simulink model "StarshipSystemModel"  (R2025b)
settings: Solver=VariableStepAuto  StartTime=0.0  StopTime=10.0  RelTol=1e-3
model workspace (MAT data in the model file):
  ActiveGNCMode : Simulink.Bus (value not decoded)
  AerodynamicControlCommand : Simulink.Bus (value not decoded)
  AerodynamicLoad : Simulink.Bus (value not decoded)
  AggregatedStream : Simulink.Bus (value not decoded)
  AllocatedEffectorDemand : Simulink.Bus (value not decoded)
  AttitudeControlDemand : Simulink.Bus (value not decoded)
  AttitudeGuidanceCommand : Simulink.Bus (value not decoded)
  AttitudeRateState : Simulink.Bus (value not decoded)
  AutogenousPressurantGas : Simulink.ConnectionBus (value not decoded)
  CandidateFaultIndication : Simulink.Bus (value not decoded)
  CombustionGasFeed : Simulink.ConnectionBus (value not decoded)
  CommandPathHealth : Simulink.Bus (value not decoded)
  ControlMode : Simulink.ValueType (value not decoded)
  DownlinkSignal : Simulink.Bus (value not decoded)
  ElectricalPower : Simulink.ConnectionBus (value not decoded)
  EngineTelemetry : Simulink.Bus (value not decoded)
  ExecutionContext : Simulink.Bus (value not decoded)
  FaultDiagnosisResult : Simulink.Bus (value not decoded)
  GNCDataContext : Simulink.Bus (value not decoded)
  GNCHealthState : Simulink.Bus (value not decoded)
  GNCStateEstimate : Simulink.Bus (value not decoded)
  GimbalAngle : Simulink.ValueType (value not decoded)
  GimbalMotion : Simulink.ConnectionBus (value not decoded)
  GroundCheckoutLink : Simulink.Bus (value not decoded)
  GroundPressurantSupply : Simulink.ConnectionBus (value not decoded)
  GuidanceConstraints : Simulink.Bus (value not decoded)
  GuidanceMode : Simulink.ValueType (value not decoded)
  LinkHealth : Simulink.Bus (value not decoded)
  LiquidPropellantFeed : Simulink.ConnectionBus (value not decoded)
  MechanicalMotion : Simulink.ConnectionBus (value not decoded)
  MechanismPosition : Simulink.Bus (value not decoded)
  ModeTransitionContext : Simulink.Bus (value not decoded)
  NavigationAidingData : Simulink.Bus (value not decoded)
  NavigationEstimate : Simulink.Bus (value not decoded)
  NavigationHealthStatus : Simulink.Bus (value not decoded)
  NavigationMeasurementSet : Simulink.Bus (value not decoded)
  PercentThrottle : Simulink.ValueType (value not decoded)
  PneumaticActuationGas : Simulink.ConnectionBus (value not decoded)
  PowerConversionStatus : Simulink.Bus (value not decoded)
  PowerDistributionStatus : Simulink.Bus (value not decoded)
  PowerHealthStatus : Simulink.Bus (value not decoded)
  PowerManagementCommand : Simulink.Bus (value not decoded)
  PowerStorageStatus : Simulink.Bus (value not decoded)
  ProtectedThermalState : Simulink.Bus (value not decoded)
  ProtectionIsolationStatus : Simulink.Bus (value not decoded)
  PurgeGasSupply : Simulink.ConnectionBus (value not decoded)
  RCSPulseCommand : Simulink.Bus (value not decoded)
  RCSTelemetry : Simulink.Bus (value not decoded)
  RFFeed : Simulink.ConnectionBus (value not decoded)
  RecoveryMechanismCommand : Simulink.Bus (value not decoded)
  RollThrottleBias : Simulink.ValueType (value not decoded)
  SafetyOverride : Simulink.ValueType (value not decoded)
  SafetyStateStatus : Simulink.Bus (value not decoded)
  ShapedControlDemand : Simulink.Bus (value not decoded)
  SpinStartIgniterGas : Simulink.ConnectionBus (value not decoded)
  StageMechanicalBoundary : Simulink.ConnectionBus (value not decoded)
  StructuralLoad : Simulink.ConnectionBus (value not decoded)
  StructureHealthStatus : Simulink.Bus (value not decoded)
  SubsystemHealthEvidence : Simulink.Bus (value not decoded)
  SubsystemStatusTelemetry : Simulink.Bus (value not decoded)
  TankTelemetry : Simulink.Bus (value not decoded)
  ThermalMonitoringCommand : Simulink.Bus (value not decoded)
  ThermalNetwork : Simulink.ConnectionBus (value not decoded)
  ThrustLoad : Simulink.ConnectionBus (value not decoded)
  TrajectoryGuidanceCommand : Simulink.Bus (value not decoded)
  TrajectoryReference : Simulink.Bus (value not decoded)
  TranslationalControlDemand : Simulink.Bus (value not decoded)
  TranslationalState : Simulink.Bus (value not decoded)
  UplinkSignal : Simulink.Bus (value not decoded)
  ValidatedControlDemand : Simulink.Bus (value not decoded)
  ValveCommand : Simulink.ValueType (value not decoded)
  VehicleStructureState : Simulink.Bus (value not decoded)
  VerifiedCommand : Simulink.Bus (value not decoded)
  VideoStream : Simulink.Bus (value not decoded)
undefined symbols (not defined in the file): ACR, ACT, ASM, ATM, BCR, BDQ, BDR, BDX, BEC, BFC, BHV, BIP, BLM, BNZ, BPI, BPR, BPV, BRX, BSM, BTA, BTP, BVC, BVE, BVV, CAA, CAM, CAS, CAT, CLM, COM, CRS, CTL, CTR, DAQ, ESC, EXT, FCR, FDB, FDE, FEX, FHI, FHM, FIC, FIS, FMG, FSC, GAP, GCM, GMD, GNC, GND, GPH, GTR, HDN, HIA, HSI, IF, INT, LOC, NAI ... (+45)
(part 2 of 8)

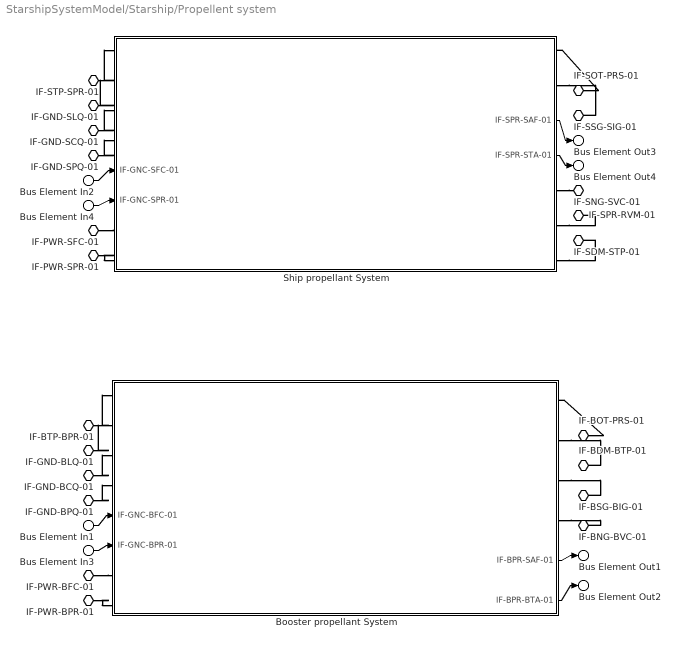
== system StarshipSystemModel/Starship/Propellent system ==
  Bus Element In1 : Inport  PortName=IF-GNC-BFC-01
  Bus Element In2 : Inport  Port=2  PortName=IF-GNC-SFC-01
  Bus Element In3 : Inport  Port=3  PortName=IF-GNC-BPR-01
  Bus Element In4 : Inport  Port=4  PortName=IF-GNC-SPR-01
  Booster propellant System : Subsystem
      settings: PortSchema="{\"entries\":[{\"content\":{\"headerSize\":26,\"margin\":15,\"minimumSpacing\":25,\"sides\":[{\"content\":{\"connectorIds\":[\"LConn2\",\"LConn3\",\"LConn4\",\"LConn7\",\"In1\",\"In2\",\"LConn5\",\"LConn6\"]},\"type\":\"ConnectorPlacement.EquallySpacedRectSide\",\"uuid\":\"fbe4f8e6-132c-4a0c-8c4c-52d0209da778\"},{\"content\":{\"connectorIds\":[\"LConn1\",\"RConn1\",\"RConn2\",\"RConn3\",\"Out1\",\"Out2\"],\"side\":\"RIGHT\"},\"type\":\"ConnectorPlacement.EquallySpacedRectSide\",\"uuid\":\"bbe80fa3-b8e3-44c5-9574-5758a55378fd\"},{\"content\":{\"side\":\"TOP\"},\"type\":\"ConnectorPlacement.EquallySpacedRectSide\",\"uuid\":\"410005e2-e10b-4d3e-a617-d51b1ea5de7e\"}]},\"type\":\"ConnectorPlacement.EquallySpacedConnector\",\"uuid\":\"b66a347a-e5b4-46b1-8a3f-28cf70f30a27\"}],\"packageUris\":[\"http://schema.mathworks.com/mf0/Connector/R2020b\"],\"version\":\"1.0\"}"
  Ship propellant System : Subsystem
      settings: PortSchema="{\"entries\":[{\"content\":{\"headerSize\":26,\"margin\":15,\"minimumSpacing\":25,\"sides\":[{\"content\":{\"connectorIds\":[\"LConn2\",\"LConn3\",\"LConn4\",\"LConn6\",\"In1\",\"In2\",\"LConn5\",\"RConn1\"]},\"type\":\"ConnectorPlacement.EquallySpacedRectSide\",\"uuid\":\"fbe4f8e6-132c-4a0c-8c4c-52d0209da778\"},{\"content\":{\"connectorIds\":[\"LConn1\",\"RConn2\",\"Out1\",\"Out2\",\"RConn3\",\"RConn4\",\"RConn5\"],\"side\":\"RIGHT\"},\"type\":\"ConnectorPlacement.EquallySpacedRectSide\",\"uuid\":\"bbe80fa3-b8e3-44c5-9574-5758a55378fd\"},{\"content\":{\"side\":\"TOP\"},\"type\":\"ConnectorPlacement.EquallySpacedRectSide\",\"uuid\":\"410005e2-e10b-4d3e-a617-d51b1ea5de7e\"},{\"content\":{\"side\":\"BOTTOM\"},\"type\":\"ConnectorPlacement.EquallySpacedRectSide\",\"uuid\":\"fc3d345f-9ee7-43d3-a8e7-80d4ac46c4c5\"}]},\"type\":\"ConnectorPlacement.EquallySpacedConnector\",\"uuid\":\"b66a347a-e5b4-46b1-8a3f-28cf70f30a27\"}],\"packageUris\":[\"http://schema.mathworks.com/mf0/Connector/R2020b\"],\"version\":\"1.0\"}"
  IF-BDM-BTP-01 : PMIOPort  Side=Right  ConnectionType=Bus: LiquidPropellantFeed
  IF-BSG-BIG-01 : PMIOPort  Port=2  Side=Right  ConnectionType=Bus: SpinStartIgniterGas
  IF-BNG-BVC-01 : PMIOPort  Port=3  Side=Right  ConnectionType=Bus: PneumaticActuationGas
  IF-SDM-STP-01 : PMIOPort  Port=4  Side=Right  ConnectionType=Bus: LiquidPropellantFeed
  IF-SPR-RVM-01 : PMIOPort  Port=5  Side=Right  ConnectionType=Bus: CombustionGasFeed
  IF-SNG-SVC-01 : PMIOPort  Port=6  Side=Right  ConnectionType=Bus: PneumaticActuationGas
  IF-SSG-SIG-01 : PMIOPort  Port=7  Side=Right  ConnectionType=Bus: SpinStartIgniterGas
  IF-BOT-PRS-01 : PMIOPort  Port=8  Side=Left  ConnectionType=Bus: StructuralLoad
  IF-SOT-PRS-01 : PMIOPort  Port=9  Side=Left  ConnectionType=Bus: StructuralLoad
  IF-BTP-BPR-01 : PMIOPort  Port=10  Side=Left  ConnectionType=Bus: AutogenousPressurantGas
  "IF-GND-BLQ-01\t" : PMIOPort  Port=11  Side=Left
  IF-STP-SPR-01 : PMIOPort  Port=12  Side=Left  ConnectionType=Bus: AutogenousPressurantGas
  "IF-GND-BCQ-01\t" : PMIOPort  Port=13  Side=Left
  IF-GND-BPQ-01 : PMIOPort  Port=14  Side=Left  ConnectionType=Bus: GroundPressurantSupply
  IF-GND-SLQ-01 : PMIOPort  Port=15  Side=Left
  IF-PWR-BFC-01 : PMIOPort  Port=16  Side=Left  ConnectionType=Bus: ElectricalPower
  IF-PWR-BPR-01 : PMIOPort  Port=17  Side=Left  ConnectionType=Bus: ElectricalPower
  IF-PWR-SFC-01 : PMIOPort  Port=18  Side=Left  ConnectionType=Bus: ElectricalPower
  IF-PWR-SPR-01 : PMIOPort  Port=19  Side=Left  ConnectionType=Bus: ElectricalPower
  IF-GND-SCQ-01 : PMIOPort  Port=20  Side=Left
  IF-GND-SPQ-01 : PMIOPort  Port=21  Side=Left  ConnectionType=Bus: GroundPressurantSupply
  Bus Element Out2 : Outport  PortName=IF-BPR-BTA-01
  Bus Element Out4 : Outport  Port=2  PortName=IF-SPR-STA-01
  Bus Element Out3 : Outport  Port=3  PortName=IF-SPR-SAF-01
  Bus Element Out1 : Outport  Port=4  PortName=IF-BPR-SAF-01
  wires:
  Booster propellant System/1(IF-BPR-SAF-01) -> Bus Element Out1/1
  Bus Element In2/1 -> Ship propellant System/1(IF-GNC-SFC-01)
  Bus Element In4/1 -> Ship propellant System/2(IF-GNC-SPR-01)
  Bus Element In3/1 -> Booster propellant System/2(IF-GNC-BPR-01)
  Bus Element In1/1 -> Booster propellant System/1(IF-GNC-BFC-01)
  Booster propellant System/2(IF-BPR-BTA-01) -> Bus Element Out2/1
  Ship propellant System/1(IF-SPR-SAF-01) -> Bus Element Out3/1
  Ship propellant System/2(IF-SPR-STA-01) -> Bus Element Out4/1
  connections:
  IF-STP-SPR-01/RConn1 -- Ship propellant System/LConn2
  IF-GND-SPQ-01/RConn1 -- Ship propellant System/LConn6
  Booster propellant System/RConn1 -- IF-BDM-BTP-01/RConn1
  IF-GND-SCQ-01/RConn1 -- Ship propellant System/LConn4
  IF-GND-SLQ-01/RConn1 -- Ship propellant System/LConn3
  IF-BTP-BPR-01/RConn1 -- Booster propellant System/LConn2
  "IF-GND-BLQ-01\t"/RConn1 -- Booster propellant System/LConn3
  "IF-GND-BCQ-01\t"/RConn1 -- Booster propellant System/LConn4
  Booster propellant System/RConn3 -- IF-BNG-BVC-01/RConn1
  IF-GND-BPQ-01/RConn1 -- Booster propellant System/LConn7
  Ship propellant System/RConn2 -- IF-SSG-SIG-01/RConn1
  Ship propellant System/RConn3 -- IF-SNG-SVC-01/RConn1
  Ship propellant System/RConn4 -- IF-SPR-RVM-01/RConn1
  Ship propellant System/RConn5 -- IF-SDM-STP-01/RConn1
  Booster propellant System/RConn2 -- IF-BSG-BIG-01/RConn1
  IF-BOT-PRS-01/RConn1 -- Booster propellant System/LConn1
  IF-SOT-PRS-01/RConn1 -- Ship propellant System/LConn1
  IF-PWR-BFC-01/RConn1 -- Booster propellant System/LConn5
  IF-PWR-BPR-01/RConn1 -- Booster propellant System/LConn6
  IF-PWR-SFC-01/RConn1 -- Ship propellant System/LConn5
  IF-PWR-SPR-01/RConn1 -- Ship propellant System/RConn1

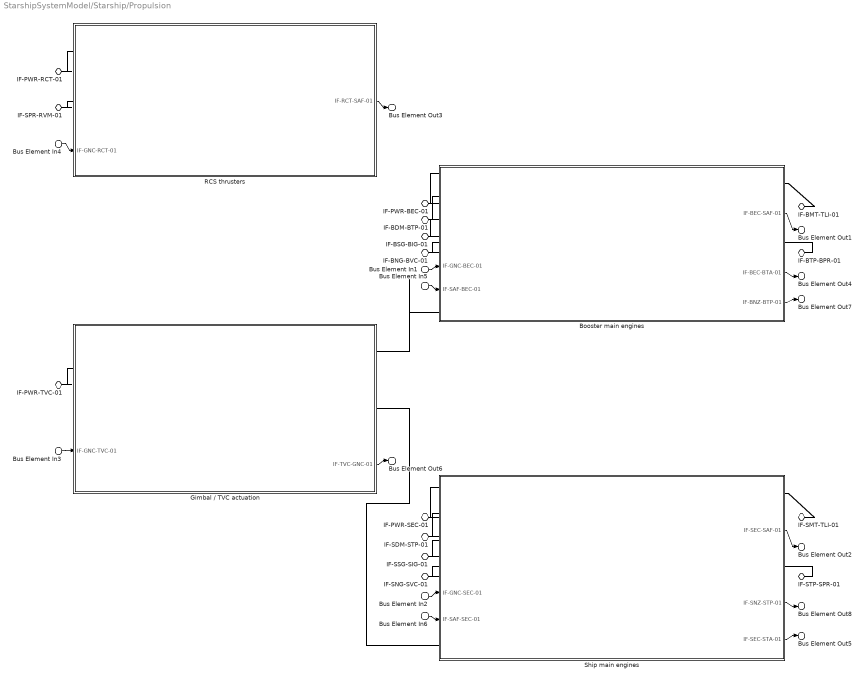
== system StarshipSystemModel/Starship/Propulsion ==
  Bus Element In1 : Inport  PortName=IF-GNC-BEC-01
  Bus Element In2 : Inport  Port=2  PortName=IF-GNC-SEC-01
  Bus Element In3 : Inport  Port=3  PortName=IF-GNC-TVC-01
  Bus Element In4 : Inport  Port=4  PortName=IF-GNC-RCT-01
  Bus Element In5 : Inport  Port=5  PortName=IF-SAF-BEC-01
  Bus Element In6 : Inport  Port=6  PortName=IF-SAF-SEC-01
  Booster main engines : Subsystem
      settings: PortSchema="{\"entries\":[{\"content\":{\"headerSize\":26,\"margin\":15,\"minimumSpacing\":25,\"sides\":[{\"content\":{\"connectorIds\":[\"LConn1\",\"LConn3\",\"LConn4\",\"LConn5\",\"In1\",\"In2\",\"LConn6\"]},\"type\":\"ConnectorPlacement.EquallySpacedRectSide\",\"uuid\":\"a24f90f9-b52e-4407-98a2-61cef3ed1001\"},{\"content\":{\"connectorIds\":[\"LConn2\",\"Out1\",\"RConn1\",\"Out2\",\"Out3\"],\"side\":\"RIGHT\"},\"type\":\"ConnectorPlacement.EquallySpacedRectSide\",\"uuid\":\"349c89d4-9966-4ad9-ba76-db4d38641e72\"},{\"content\":{\"side\":\"TOP\"},\"type\":\"ConnectorPlacement.EquallySpacedRectSide\",\"uuid\":\"c23b8a3e-5693-4bb4-96b3-90d999333c4e\"}]},\"type\":\"ConnectorPlacement.EquallySpacedConnector\",\"uuid\":\"ab682651-c32f-4460-8c4f-01dcf64563ad\"}],\"packageUris\":[\"http://schema.mathworks.com/mf0/Connector/R2020b\"],\"version\":\"1.0\"}"
  Gimbal / TVC actuation : Subsystem
      settings: PortSchema="{\"entries\":[{\"content\":{\"headerSize\":26,\"margin\":15,\"minimumSpacing\":25,\"sides\":[{\"content\":{\"connectorIds\":[\"LConn1\",\"In1\"]},\"type\":\"ConnectorPlacement.EquallySpacedRectSide\",\"uuid\":\"a24f90f9-b52e-4407-98a2-61cef3ed1001\"},{\"content\":{\"connectorIds\":[\"RConn1\",\"RConn2\",\"Out1\"],\"side\":\"RIGHT\"},\"type\":\"ConnectorPlacement.EquallySpacedRectSide\",\"uuid\":\"349c89d4-9966-4ad9-ba76-db4d38641e72\"},{\"content\":{\"side\":\"TOP\"},\"type\":\"ConnectorPlacement.EquallySpacedRectSide\",\"uuid\":\"c23b8a3e-5693-4bb4-96b3-90d999333c4e\"}]},\"type\":\"ConnectorPlacement.EquallySpacedConnector\",\"uuid\":\"ab682651-c32f-4460-8c4f-01dcf64563ad\"}],\"packageUris\":[\"http://schema.mathworks.com/mf0/Connector/R2020b\"],\"version\":\"1.0\"}"
  RCS thrusters : Subsystem
      settings: PortSchema="{\"entries\":[{\"content\":{\"headerSize\":26,\"margin\":15,\"minimumSpacing\":25,\"sides\":[{\"content\":{\"connectorIds\":[\"LConn1\",\"LConn2\",\"In1\"]},\"type\":\"ConnectorPlacement.EquallySpacedRectSide\",\"uuid\":\"a24f90f9-b52e-4407-98a2-61cef3ed1001\"},{\"content\":{\"connectorIds\":[\"Out1\"],\"side\":\"RIGHT\"},\"type\":\"ConnectorPlacement.EquallySpacedRectSide\",\"uuid\":\"349c89d4-9966-4ad9-ba76-db4d38641e72\"},{\"content\":{\"side\":\"TOP\"},\"type\":\"ConnectorPlacement.EquallySpacedRectSide\",\"uuid\":\"c23b8a3e-5693-4bb4-96b3-90d999333c4e\"}]},\"type\":\"ConnectorPlacement.EquallySpacedConnector\",\"uuid\":\"ab682651-c32f-4460-8c4f-01dcf64563ad\"}],\"packageUris\":[\"http://schema.mathworks.com/mf0/Connector/R2020b\"],\"version\":\"1.0\"}"
  Ship main engines : Subsystem
      settings: PortSchema="{\"entries\":[{\"content\":{\"headerSize\":26,\"margin\":15,\"minimumSpacing\":25,\"sides\":[{\"content\":{\"connectorIds\":[\"LConn1\",\"LConn3\",\"LConn4\",\"LConn5\",\"In1\",\"In2\",\"LConn6\"]},\"type\":\"ConnectorPlacement.EquallySpacedRectSide\",\"uuid\":\"a24f90f9-b52e-4407-98a2-61cef3ed1001\"},{\"content\":{\"connectorIds\":[\"LConn2\",\"Out1\",\"RConn1\",\"Out2\",\"Out3\"],\"side\":\"RIGHT\"},\"type\":\"ConnectorPlacement.EquallySpacedRectSide\",\"uuid\":\"349c89d4-9966-4ad9-ba76-db4d38641e72\"},{\"content\":{\"side\":\"TOP\"},\"type\":\"ConnectorPlacement.EquallySpacedRectSide\",\"uuid\":\"c23b8a3e-5693-4bb4-96b3-90d999333c4e\"}]},\"type\":\"ConnectorPlacement.EquallySpacedConnector\",\"uuid\":\"ab682651-c32f-4460-8c4f-01dcf64563ad\"}],\"packageUris\":[\"http://schema.mathworks.com/mf0/Connector/R2020b\"],\"version\":\"1.0\"}"
  IF-PWR-RCT-01 : PMIOPort  Side=Left  ConnectionType=Bus: ElectricalPower
  IF-PWR-TVC-01 : PMIOPort  Port=2  Side=Left  ConnectionType=Bus: ElectricalPower
  IF-PWR-BEC-01 : PMIOPort  Port=3  Side=Left  ConnectionType=Bus: ElectricalPower
  IF-PWR-SEC-01 : PMIOPort  Port=4  Side=Left  ConnectionType=Bus: ElectricalPower
  IF-BMT-TLI-01 : PMIOPort  Port=5  Side=Left  ConnectionType=Bus: StructuralLoad
  IF-SMT-TLI-01 : PMIOPort  Port=6  Side=Left  ConnectionType=Bus: StructuralLoad
  IF-BDM-BTP-01 : PMIOPort  Port=7  Side=Left  ConnectionType=Bus: LiquidPropellantFeed
  IF-SDM-STP-01 : PMIOPort  Port=8  Side=Left  ConnectionType=Bus: LiquidPropellantFeed
  IF-SPR-RVM-01 : PMIOPort  Port=9  Side=Left  ConnectionType=Bus: CombustionGasFeed
  IF-BSG-BIG-01 : PMIOPort  Port=10  Side=Left  ConnectionType=Bus: SpinStartIgniterGas
  IF-BNG-BVC-01 : PMIOPort  Port=11  Side=Left  ConnectionType=Bus: PneumaticActuationGas
  IF-SSG-SIG-01 : PMIOPort  Port=12  Side=Left  ConnectionType=Bus: SpinStartIgniterGas
  IF-SNG-SVC-01 : PMIOPort  Port=13  Side=Left  ConnectionType=Bus: PneumaticActuationGas
  IF-BTP-BPR-01 : PMIOPort  Port=14  Side=Right  ConnectionType=Bus: AutogenousPressurantGas
  IF-STP-SPR-01 : PMIOPort  Port=15  Side=Right  ConnectionType=Bus: AutogenousPressurantGas
  Bus Element Out3 : Outport  PortName=IF-RCT-SAF-01
  Bus Element Out4 : Outport  Port=2  PortName=IF-BEC-BTA-01
  Bus Element Out7 : Outport  Port=3  PortName=IF-BNZ-BTP-01
  Bus Element Out1 : Outport  Port=4  PortName=IF-BEC-SAF-01
  Bus Element Out6 : Outport  Port=5  PortName=IF-TVC-GNC-01
  Bus Element Out5 : Outport  Port=6  PortName=IF-SEC-STA-01
  Bus Element Out2 : Outport  Port=7  PortName=IF-SEC-SAF-01
  Bus Element Out8 : Outport  Port=8  PortName=IF-SNZ-STP-01
  wires:
  RCS thrusters/1(IF-RCT-SAF-01) -> Bus Element Out3/1
  Bus Element In6/1 -> Ship main engines/2(IF-SAF-SEC-01)
  Bus Element In5/1 -> Booster main engines/2(IF-SAF-BEC-01)
  Bus Element In4/1 -> RCS thrusters/1(IF-GNC-RCT-01)
  Bus Element In3/1 -> Gimbal / TVC actuation/1(IF-GNC-TVC-01)
  Bus Element In2/1 -> Ship main engines/1(IF-GNC-SEC-01)
  Gimbal / TVC actuation/1(IF-TVC-GNC-01) -> Bus Element Out6/1
  Bus Element In1/1 -> Booster main engines/1(IF-GNC-BEC-01)
  Booster main engines/1(IF-BEC-SAF-01) -> Bus Element Out1/1
  Booster main engines/2(IF-BEC-BTA-01) -> Bus Element Out4/1
  Ship main engines/1(IF-SEC-SAF-01) -> Bus Element Out2/1
  Ship main engines/3(IF-SEC-STA-01) -> Bus Element Out5/1
  Booster main engines/3(IF-BNZ-BTP-01) -> Bus Element Out7/1
  Ship main engines/2(IF-SNZ-STP-01) -> Bus Element Out8/1
  connections:
  IF-SPR-RVM-01/RConn1 -- RCS thrusters/LConn2
  IF-BDM-BTP-01/RConn1 -- Booster main engines/LConn3
  IF-SDM-STP-01/RConn1 -- Ship main engines/LConn3
  Gimbal / TVC actuation/RConn1 -- Booster main engines/LConn6
  Gimbal / TVC actuation/RConn2 -- Ship main engines/LConn6
  IF-BSG-BIG-01/RConn1 -- Booster main engines/LConn4
  IF-BNG-BVC-01/RConn1 -- Booster main engines/LConn5
  IF-SSG-SIG-01/RConn1 -- Ship main engines/LConn4
  IF-SNG-SVC-01/RConn1 -- Ship main engines/LConn5
  Booster main engines/RConn1 -- IF-BTP-BPR-01/RConn1
  Ship main engines/RConn1 -- IF-STP-SPR-01/RConn1
  IF-BMT-TLI-01/RConn1 -- Booster main engines/LConn2
  IF-SMT-TLI-01/RConn1 -- Ship main engines/LConn2
  IF-PWR-BEC-01/RConn1 -- Booster main engines/LConn1
  IF-PWR-SEC-01/RConn1 -- Ship main engines/LConn1
  IF-PWR-TVC-01/RConn1 -- Gimbal / TVC actuation/LConn1
  IF-PWR-RCT-01/RConn1 -- RCS thrusters/LConn1

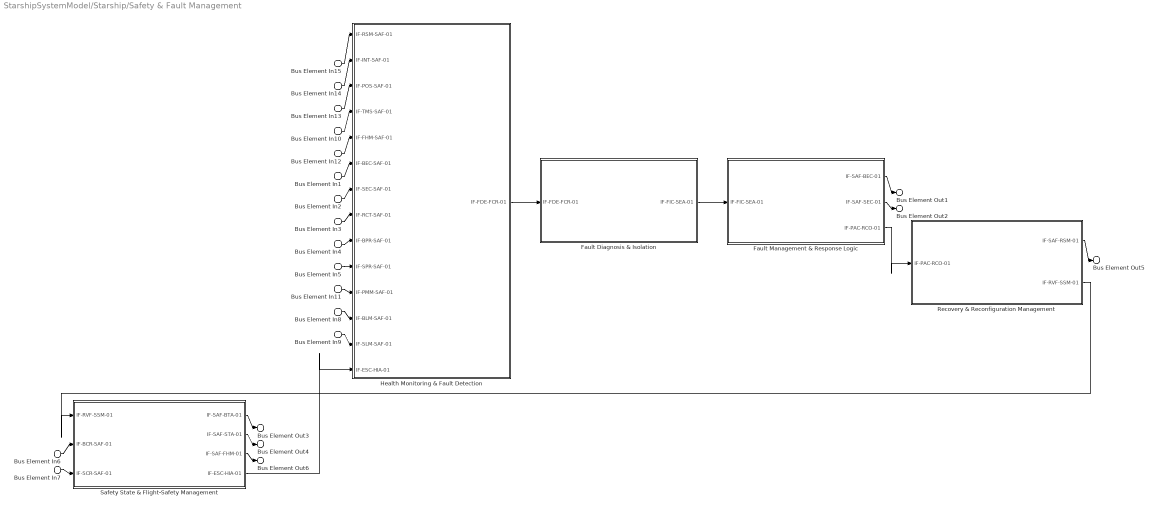
== system StarshipSystemModel/Starship/Safety & Fault Management  ==
  Bus Element In15 : Inport  PortName=IF-RSM-SAF-01
  Bus Element In14 : Inport  Port=2  PortName=IF-INT-SAF-01
  Bus Element In13 : Inport  Port=3  PortName=IF-POS-SAF-01
  Bus Element In12 : Inport  Port=4  PortName=IF-FHM-SAF-01
  Bus Element In11 : Inport  Port=5  PortName=IF-PMM-SAF-01
  Bus Element In10 : Inport  Port=6  PortName=IF-TMS-SAF-01
  Bus Element In5 : Inport  Port=7  PortName=IF-SPR-SAF-01
  Bus Element In4 : Inport  Port=8  PortName=IF-BPR-SAF-01
  Bus Element In1 : Inport  Port=9  PortName=IF-BEC-SAF-01
  Bus Element In3 : Inport  Port=10  PortName=IF-RCT-SAF-01
  Bus Element In2 : Inport  Port=11  PortName=IF-SEC-SAF-01
  Bus Element In6 : Inport  Port=12  PortName=IF-BCR-SAF-01
  Bus Element In7 : Inport  Port=13  PortName=IF-SCR-SAF-01
  Bus Element In8 : Inport  Port=14  PortName=IF-BLM-SAF-01
  Bus Element In9 : Inport  Port=15  PortName=IF-SLM-SAF-01
  Fault Diagnosis & Isolation : Subsystem
      settings: PortSchema="{\"entries\":[{\"content\":{\"headerSize\":26,\"margin\":15,\"minimumSpacing\":25,\"sides\":[{\"content\":{\"connectorIds\":[\"In1\"]},\"type\":\"ConnectorPlacement.EquallySpacedRectSide\",\"uuid\":\"c1b9b7ae-a5d1-4a08-a561-f06fbe6dc300\"},{\"content\":{\"connectorIds\":[\"Out1\"],\"side\":\"RIGHT\"},\"type\":\"ConnectorPlacement.EquallySpacedRectSide\",\"uuid\":\"af8a3603-108a-44dc-af3d-660c23f2553a\"},{\"content\":{\"side\":\"TOP\"},\"type\":\"ConnectorPlacement.EquallySpacedRectSide\",\"uuid\":\"59101f68-40fe-4ccb-9258-ad0f93699a98\"}]},\"type\":\"ConnectorPlacement.EquallySpacedConnector\",\"uuid\":\"683df2e7-6d18-4135-a0d1-7e7a3e3475d2\"}],\"packageUris\":[\"http://schema.mathworks.com/mf0/Connector/R2020b\"],\"version\":\"1.0\"}"
  Fault Management & Response Logic : Subsystem
      settings: PortSchema="{\"entries\":[{\"content\":{\"headerSize\":26,\"margin\":15,\"minimumSpacing\":25,\"sides\":[{\"content\":{\"connectorIds\":[\"In1\"]},\"type\":\"ConnectorPlacement.EquallySpacedRectSide\",\"uuid\":\"c1b9b7ae-a5d1-4a08-a561-f06fbe6dc300\"},{\"content\":{\"connectorIds\":[\"Out1\",\"Out2\",\"Out3\"],\"side\":\"RIGHT\"},\"type\":\"ConnectorPlacement.EquallySpacedRectSide\",\"uuid\":\"af8a3603-108a-44dc-af3d-660c23f2553a\"},{\"content\":{\"side\":\"TOP\"},\"type\":\"ConnectorPlacement.EquallySpacedRectSide\",\"uuid\":\"59101f68-40fe-4ccb-9258-ad0f93699a98\"}]},\"type\":\"ConnectorPlacement.EquallySpacedConnector\",\"uuid\":\"683df2e7-6d18-4135-a0d1-7e7a3e3475d2\"}],\"packageUris\":[\"http://schema.mathworks.com/mf0/Connector/R2020b\"],\"version\":\"1.0\"}"
  Health Monitoring & Fault Detection : Subsystem
      settings: PortSchema="{\"entries\":[{\"content\":{\"headerSize\":26,\"margin\":15,\"minimumSpacing\":25,\"sides\":[{\"content\":{\"connectorIds\":[\"In1\",\"In2\",\"In3\",\"In4\",\"In5\",\"In6\",\"In7\",\"In8\",\"In9\",\"In10\",\"In11\",\"In12\",\"In13\",\"In14\"]},\"type\":\"ConnectorPlacement.EquallySpacedRectSide\",\"uuid\":\"c1b9b7ae-a5d1-4a08-a561-f06fbe6dc300\"},{\"content\":{\"connectorIds\":[\"Out1\"],\"side\":\"RIGHT\"},\"type\":\"ConnectorPlacement.EquallySpacedRectSide\",\"uuid\":\"af8a3603-108a-44dc-af3d-660c23f2553a\"},{\"content\":{\"side\":\"TOP\"},\"type\":\"ConnectorPlacement.EquallySpacedRectSide\",\"uuid\":\"59101f68-40fe-4ccb-9258-ad0f93699a98\"}]},\"type\":\"ConnectorPlacement.EquallySpacedConnector\",\"uuid\":\"683df2e7-6d18-4135-a0d1-7e7a3e3475d2\"}],\"packageUris\":[\"http://schema.mathworks.com/mf0/Connector/R2020b\"],\"version\":\"1.0\"}"
  Recovery & Reconfiguration Management : Subsystem
      settings: PortSchema="{\"entries\":[{\"content\":{\"headerSize\":26,\"margin\":15,\"minimumSpacing\":25,\"sides\":[{\"content\":{\"connectorIds\":[\"In1\"]},\"type\":\"ConnectorPlacement.EquallySpacedRectSide\",\"uuid\":\"c1b9b7ae-a5d1-4a08-a561-f06fbe6dc300\"},{\"content\":{\"connectorIds\":[\"Out1\",\"Out2\"],\"side\":\"RIGHT\"},\"type\":\"ConnectorPlacement.EquallySpacedRectSide\",\"uuid\":\"af8a3603-108a-44dc-af3d-660c23f2553a\"},{\"content\":{\"side\":\"TOP\"},\"type\":\"ConnectorPlacement.EquallySpacedRectSide\",\"uuid\":\"59101f68-40fe-4ccb-9258-ad0f93699a98\"}]},\"type\":\"ConnectorPlacement.EquallySpacedConnector\",\"uuid\":\"683df2e7-6d18-4135-a0d1-7e7a3e3475d2\"}],\"packageUris\":[\"http://schema.mathworks.com/mf0/Connector/R2020b\"],\"version\":\"1.0\"}"
  Safety State & Flight-Safety Management : Subsystem
      settings: PortSchema="{\"entries\":[{\"content\":{\"headerSize\":26,\"margin\":15,\"minimumSpacing\":25,\"sides\":[{\"content\":{\"connectorIds\":[\"In1\",\"In2\",\"In3\"]},\"type\":\"ConnectorPlacement.EquallySpacedRectSide\",\"uuid\":\"c1b9b7ae-a5d1-4a08-a561-f06fbe6dc300\"},{\"content\":{\"connectorIds\":[\"Out1\",\"Out2\",\"Out3\",\"Out4\"],\"side\":\"RIGHT\"},\"type\":\"ConnectorPlacement.EquallySpacedRectSide\",\"uuid\":\"af8a3603-108a-44dc-af3d-660c23f2553a\"},{\"content\":{\"side\":\"TOP\"},\"type\":\"ConnectorPlacement.EquallySpacedRectSide\",\"uuid\":\"59101f68-40fe-4ccb-9258-ad0f93699a98\"}]},\"type\":\"ConnectorPlacement.EquallySpacedConnector\",\"uuid\":\"683df2e7-6d18-4135-a0d1-7e7a3e3475d2\"}],\"packageUris\":[\"http://schema.mathworks.com/mf0/Connector/R2020b\"],\"version\":\"1.0\"}"
  Bus Element Out5 : Outport  PortName=IF-SAF-RSM-01
  Bus Element Out2 : Outport  Port=2  PortName=IF-SAF-SEC-01
  Bus Element Out3 : Outport  Port=3  PortName=IF-SAF-BTA-01
  Bus Element Out1 : Outport  Port=4  PortName=IF-SAF-BEC-01
  Bus Element Out4 : Outport  Port=5  PortName=IF-SAF-STA-01
  Bus Element Out6 : Outport  Port=6  PortName=IF-SAF-FHM-01
  wires:
  Bus Element In12/1 -> Health Monitoring & Fault Detection/5(IF-FHM-SAF-01)
  Bus Element In10/1 -> Health Monitoring & Fault Detection/4(IF-TMS-SAF-01)
  Bus Element In6/1 -> Safety State & Flight-Safety Management/2(IF-BCR-SAF-01)
  Bus Element In1/1 -> Health Monitoring & Fault Detection/6(IF-BEC-SAF-01)
  Bus Element In7/1 -> Safety State & Flight-Safety Management/3(IF-SCR-SAF-01)
  Bus Element In15/1 -> Health Monitoring & Fault Detection/1(IF-RSM-SAF-01)
  Bus Element In14/1 -> Health Monitoring & Fault Detection/2(IF-INT-SAF-01)
  Safety State & Flight-Safety Management/3(IF-SAF-FHM-01) -> Bus Element Out6/1
  Bus Element In13/1 -> Health Monitoring & Fault Detection/3(IF-POS-SAF-01)
  Bus Element In2/1 -> Health Monitoring & Fault Detection/7(IF-SEC-SAF-01)
  Bus Element In3/1 -> Health Monitoring & Fault Detection/8(IF-RCT-SAF-01)
  Bus Element In4/1 -> Health Monitoring & Fault Detection/9(IF-BPR-SAF-01)
  Bus Element In5/1 -> Health Monitoring & Fault Detection/10(IF-SPR-SAF-01)
  Fault Management & Response Logic/2(IF-SAF-SEC-01) -> Bus Element Out2/1
  Bus Element In11/1 -> Health Monitoring & Fault Detection/11(IF-PMM-SAF-01)
  Fault Diagnosis & Isolation/1(IF-FIC-SEA-01) -> Fault Management & Response Logic/1(IF-FIC-SEA-01)
  Bus Element In8/1 -> Health Monitoring & Fault Detection/12(IF-BLM-SAF-01)
  Bus Element In9/1 -> Health Monitoring & Fault Detection/13(IF-SLM-SAF-01)
  Safety State & Flight-Safety Management/1(IF-SAF-BTA-01) -> Bus Element Out3/1
  Safety State & Flight-Safety Management/2(IF-SAF-STA-01) -> Bus Element Out4/1
  Safety State & Flight-Safety Management/4(IF-ESC-HIA-01) -> Health Monitoring & Fault Detection/14(IF-ESC-HIA-01)
  Health Monitoring & Fault Detection/1(IF-FDE-FCR-01) -> Fault Diagnosis & Isolation/1(IF-FDE-FCR-01)
  Fault Management & Response Logic/1(IF-SAF-BEC-01) -> Bus Element Out1/1
  Fault Management & Response Logic/3(IF-PAC-RCO-01) -> Recovery & Reconfiguration Management/1(IF-PAC-RCO-01)
  Recovery & Reconfiguration Management/1(IF-SAF-RSM-01) -> Bus Element Out5/1
  Recovery & Reconfiguration Management/2(IF-RVF-SSM-01) -> Safety State & Flight-Safety Management/1(IF-RVF-SSM-01)

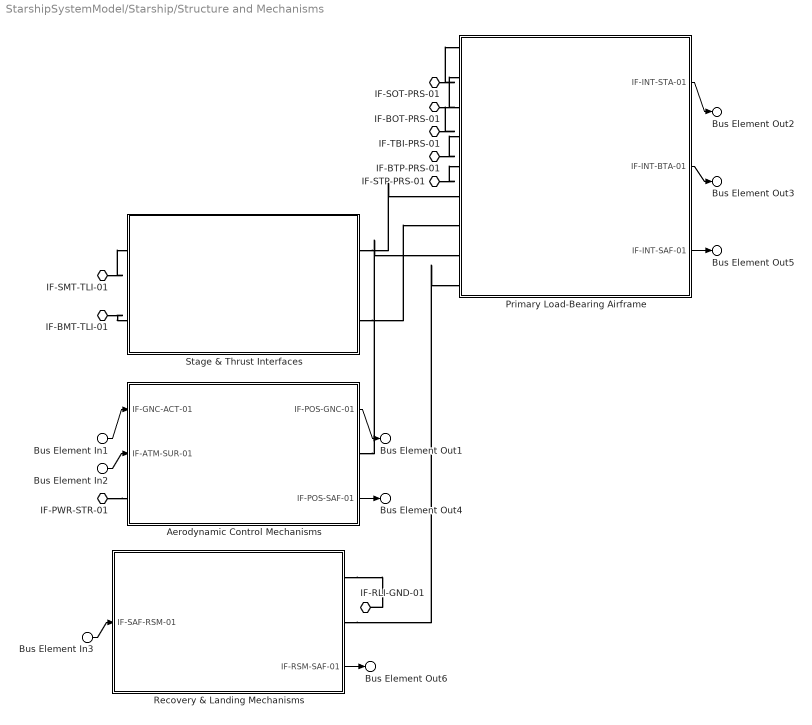
== system StarshipSystemModel/Starship/Structure and Mechanisms ==
  Bus Element In1 : Inport  PortName=IF-GNC-ACT-01
  Bus Element In2 : Inport  Port=2  PortName=IF-ATM-SUR-01
  Bus Element In3 : Inport  Port=3  PortName=IF-SAF-RSM-01
  Aerodynamic Control Mechanisms : Subsystem
      settings: PortSchema="{\"entries\":[{\"content\":{\"headerSize\":26,\"margin\":15,\"minimumSpacing\":25,\"sides\":[{\"content\":{\"connectorIds\":[\"In1\",\"In2\",\"LConn1\"]},\"type\":\"ConnectorPlacement.EquallySpacedRectSide\",\"uuid\":\"23792f18-2863-4199-9730-8799d4a474a5\"},{\"content\":{\"connectorIds\":[\"Out1\",\"RConn1\",\"Out2\"],\"side\":\"RIGHT\"},\"type\":\"ConnectorPlacement.EquallySpacedRectSide\",\"uuid\":\"c8cda51b-7b41-45d2-a922-70343296893f\"},{\"content\":{\"side\":\"TOP\"},\"type\":\"ConnectorPlacement.EquallySpacedRectSide\",\"uuid\":\"3580f4a1-1924-4d7f-ad03-70e3a97c03ce\"}]},\"type\":\"ConnectorPlacement.EquallySpacedConnector\",\"uuid\":\"f1529067-176f-4d7b-82ef-d3d6162373fd\"}],\"packageUris\":[\"http://schema.mathworks.com/mf0/Connector/R2020b\"],\"version\":\"1.0\"}"
  Primary Load-Bearing Airframe : Subsystem
      settings: PortSchema="{\"entries\":[{\"content\":{\"headerSize\":26,\"margin\":15,\"minimumSpacing\":25,\"sides\":[{\"content\":{\"connectorIds\":[\"RConn3\",\"RConn2\",\"LConn1\",\"LConn2\",\"LConn3\",\"RConn1\",\"LConn5\",\"LConn4\",\"LConn6\"]},\"type\":\"ConnectorPlacement.EquallySpacedRectSide\",\"uuid\":\"23792f18-2863-4199-9730-8799d4a474a5\"},{\"content\":{\"connectorIds\":[\"Out1\",\"Out2\",\"Out3\"],\"side\":\"RIGHT\"},\"type\":\"ConnectorPlacement.EquallySpacedRectSide\",\"uuid\":\"c8cda51b-7b41-45d2-a922-70343296893f\"},{\"content\":{\"side\":\"TOP\"},\"type\":\"ConnectorPlacement.EquallySpacedRectSide\",\"uuid\":\"3580f4a1-1924-4d7f-ad03-70e3a97c03ce\"},{\"content\":{\"side\":\"BOTTOM\"},\"type\":\"ConnectorPlacement.EquallySpacedRectSide\",\"uuid\":\"50285ac1-0d11-40d3-9d33-3131f6ed844a\"}]},\"type\":\"ConnectorPlacement.EquallySpacedConnector\",\"uuid\":\"f1529067-176f-4d7b-82ef-d3d6162373fd\"}],\"packageUris\":[\"http://schema.mathworks.com/mf0/Connector/R2020b\"],\"version\":\"1.0\"}"
  Recovery & Landing Mechanisms : Subsystem
      settings: PortSchema="{\"entries\":[{\"content\":{\"headerSize\":26,\"margin\":15,\"minimumSpacing\":25,\"sides\":[{\"content\":{\"connectorIds\":[\"In1\"]},\"type\":\"ConnectorPlacement.EquallySpacedRectSide\",\"uuid\":\"23792f18-2863-4199-9730-8799d4a474a5\"},{\"content\":{\"connectorIds\":[\"RConn1\",\"RConn2\",\"Out1\"],\"side\":\"RIGHT\"},\"type\":\"ConnectorPlacement.EquallySpacedRectSide\",\"uuid\":\"c8cda51b-7b41-45d2-a922-70343296893f\"},{\"content\":{\"side\":\"TOP\"},\"type\":\"ConnectorPlacement.EquallySpacedRectSide\",\"uuid\":\"3580f4a1-1924-4d7f-ad03-70e3a97c03ce\"}]},\"type\":\"ConnectorPlacement.EquallySpacedConnector\",\"uuid\":\"f1529067-176f-4d7b-82ef-d3d6162373fd\"}],\"packageUris\":[\"http://schema.mathworks.com/mf0/Connector/R2020b\"],\"version\":\"1.0\"}"
  Stage & Thrust Interfaces : Subsystem
      settings: PortSchema="{\"entries\":[{\"content\":{\"headerSize\":26,\"margin\":15,\"minimumSpacing\":25,\"sides\":[{\"content\":{\"connectorIds\":[\"RConn2\",\"RConn1\"]},\"type\":\"ConnectorPlacement.EquallySpacedRectSide\",\"uuid\":\"23792f18-2863-4199-9730-8799d4a474a5\"},{\"content\":{\"connectorIds\":[\"RConn3\",\"RConn4\"],\"side\":\"RIGHT\"},\"type\":\"ConnectorPlacement.EquallySpacedRectSide\",\"uuid\":\"c8cda51b-7b41-45d2-a922-70343296893f\"},{\"content\":{\"side\":\"TOP\"},\"type\":\"ConnectorPlacement.EquallySpacedRectSide\",\"uuid\":\"3580f4a1-1924-4d7f-ad03-70e3a97c03ce\"}]},\"type\":\"ConnectorPlacement.EquallySpacedConnector\",\"uuid\":\"f1529067-176f-4d7b-82ef-d3d6162373fd\"}],\"packageUris\":[\"http://schema.mathworks.com/mf0/Connector/R2020b\"],\"version\":\"1.0\"}"
  IF-BMT-TLI-01 : PMIOPort  Side=Right  ConnectionType=Bus: StructuralLoad
  IF-SMT-TLI-01 : PMIOPort  Port=2  Side=Right  ConnectionType=Bus: StructuralLoad
  IF-SOT-PRS-01 : PMIOPort  Port=3  Side=Right  ConnectionType=Bus: StructuralLoad
  IF-BOT-PRS-01 : PMIOPort  Port=4  Side=Right  ConnectionType=Bus: StructuralLoad
  IF-TBI-PRS-01 : PMIOPort  Port=5  Side=Left  ConnectionType=Bus: ThermalNetwork
  IF-BTP-PRS-01 : PMIOPort  Port=6  Side=Left  ConnectionType=Bus: ThermalNetwork
  IF-STP-PRS-01 : PMIOPort  Port=7  Side=Left  ConnectionType=Bus: ThermalNetwork
  IF-RLI-GND-01 : PMIOPort  Port=8  Side=Right  ConnectionType=Bus: StructuralLoad
  IF-PWR-STR-01 : PMIOPort  Port=9  Side=Left  ConnectionType=Bus: ElectricalPower
  Bus Element Out1 : Outport  PortName=IF-POS-GNC-01
  Bus Element Out2 : Outport  Port=2  PortName=IF-INT-STA-01
  Bus Element Out3 : Outport  Port=3  PortName=IF-INT-BTA-01
  Bus Element Out4 : Outport  Port=4  PortName=IF-POS-SAF-01
  Bus Element Out5 : Outport  Port=5  PortName=IF-INT-SAF-01
  Bus Element Out6 : Outport  Port=6  PortName=IF-RSM-SAF-01
  wires:
  Primary Load-Bearing Airframe/2(IF-INT-BTA-01) -> Bus Element Out3/1
  Bus Element In1/1 -> Aerodynamic Control Mechanisms/1(IF-GNC-ACT-01)
  Bus Element In2/1 -> Aerodynamic Control Mechanisms/2(IF-ATM-SUR-01)
  Aerodynamic Control Mechanisms/1(IF-POS-GNC-01) -> Bus Element Out1/1
  Primary Load-Bearing Airframe/1(IF-INT-STA-01) -> Bus Element Out2/1
  Aerodynamic Control Mechanisms/2(IF-POS-SAF-01) -> Bus Element Out4/1
  Primary Load-Bearing Airframe/3(IF-INT-SAF-01) -> Bus Element Out5/1
  Recovery & Landing Mechanisms/1(IF-RSM-SAF-01) -> Bus Element Out6/1
  Bus Element In3/1 -> Recovery & Landing Mechanisms/1(IF-SAF-RSM-01)
  connections:
  IF-BOT-PRS-01/RConn1 -- Primary Load-Bearing Airframe/RConn2
  IF-SMT-TLI-01/RConn1 -- Stage & Thrust Interfaces/RConn2
  IF-SOT-PRS-01/RConn1 -- Primary Load-Bearing Airframe/RConn3
  IF-BMT-TLI-01/RConn1 -- Stage & Thrust Interfaces/RConn1
  IF-TBI-PRS-01/RConn1 -- Primary Load-Bearing Airframe/LConn1
  Stage & Thrust Interfaces/RConn4 -- Primary Load-Bearing Airframe/LConn5
  IF-BTP-PRS-01/RConn1 -- Primary Load-Bearing Airframe/LConn2
  IF-STP-PRS-01/RConn1 -- Primary Load-Bearing Airframe/LConn3
  Stage & Thrust Interfaces/RConn3 -- Primary Load-Bearing Airframe/RConn1
  Aerodynamic Control Mechanisms/RConn1 -- Primary Load-Bearing Airframe/LConn4
  Recovery & Landing Mechanisms/RConn1 -- IF-RLI-GND-01/RConn1
  Recovery & Landing Mechanisms/RConn2 -- Primary Load-Bearing Airframe/LConn6
  IF-PWR-STR-01/RConn1 -- Aerodynamic Control Mechanisms/LConn1

== system StarshipSystemModel/Starship/Thermal Protection ==
  Bus Element In5 : Inport  PortName=IF-GNC-TMS-01
  Bus Element In4 : Inport  Port=2  PortName=IF-SNZ-STP-01
  Bus Element In3 : Inport  Port=3  PortName=IF-BNZ-BTP-01
  Bus Element In1 : Inport  Port=4  PortName=IF-ATM-STP-01
  Bus Element In2 : Inport  Port=5  PortName=IF-ATM-BTP-01
  Ship Primary TPS : Subsystem
      settings: PortSchema="{\"entries\":[{\"content\":{\"headerSize\":26,\"margin\":15,\"minimumSpacing\":25,\"sides\":[{\"content\":{\"connectorIds\":[\"In1\",\"In2\"]},\"type\":\"ConnectorPlacement.EquallySpacedRectSide\",\"uuid\":\"e0cfb70a-2480-46ad-8838-78efdb61b60e\"},{\"content\":{\"connectorIds\":[\"RConn1\",\"Out1\",\"Out2\",\"Out3\"],\"side\":\"RIGHT\"},\"type\":\"ConnectorPlacement.EquallySpacedRectSide\",\"uuid\":\"0844e172-3ed8-42bd-94dc-a51d08e37039\"},{\"content\":{\"side\":\"TOP\"},\"type\":\"ConnectorPlacement.EquallySpacedRectSide\",\"uuid\":\"2415ea6e-ae7d-422f-a1cc-5a10cd0c87f7\"}]},\"type\":\"ConnectorPlacement.EquallySpacedConnector\",\"uuid\":\"814347a2-9201-4b2d-b96f-a93fca4a3c45\"}],\"packageUris\":[\"http://schema.mathworks.com/mf0/Connector/R2020b\"],\"version\":\"1.0\"}"
  Super Heavy Thermal Protection : Subsystem
      settings: PortSchema="{\"entries\":[{\"content\":{\"headerSize\":26,\"margin\":15,\"minimumSpacing\":25,\"sides\":[{\"content\":{\"connectorIds\":[\"In1\",\"In2\"]},\"type\":\"ConnectorPlacement.EquallySpacedRectSide\",\"uuid\":\"e0cfb70a-2480-46ad-8838-78efdb61b60e\"},{\"content\":{\"connectorIds\":[\"Out1\",\"Out2\",\"Out3\",\"RConn1\"],\"side\":\"RIGHT\"},\"type\":\"ConnectorPlacement.EquallySpacedRectSide\",\"uuid\":\"0844e172-3ed8-42bd-94dc-a51d08e37039\"},{\"content\":{\"side\":\"TOP\"},\"type\":\"ConnectorPlacement.EquallySpacedRectSide\",\"uuid\":\"2415ea6e-ae7d-422f-a1cc-5a10cd0c87f7\"}]},\"type\":\"ConnectorPlacement.EquallySpacedConnector\",\"uuid\":\"814347a2-9201-4b2d-b96f-a93fca4a3c45\"}],\"packageUris\":[\"http://schema.mathworks.com/mf0/Connector/R2020b\"],\"version\":\"1.0\"}"
  Thermal Barriers & Discontinuity Protection : Subsystem
      settings: PortSchema="{\"entries\":[{\"content\":{\"headerSize\":26,\"margin\":15,\"minimumSpacing\":25,\"sides\":[{\"content\":{\"connectorIds\":[\"In1\",\"In2\",\"In3\",\"In4\",\"In5\",\"In6\"]},\"type\":\"ConnectorPlacement.EquallySpacedRectSide\",\"uuid\":\"e0cfb70a-2480-46ad-8838-78efdb61b60e\"},{\"content\":{\"connectorIds\":[\"Out1\",\"Out2\",\"Out3\",\"RConn1\"],\"side\":\"RIGHT\"},\"type\":\"ConnectorPlacement.EquallySpacedRectSide\",\"uuid\":\"0844e172-3ed8-42bd-94dc-a51d08e37039\"},{\"content\":{\"side\":\"TOP\"},\"type\":\"ConnectorPlacement.EquallySpacedRectSide\",\"uuid\":\"2415ea6e-ae7d-422f-a1cc-5a10cd0c87f7\"}]},\"type\":\"ConnectorPlacement.EquallySpacedConnector\",\"uuid\":\"814347a2-9201-4b2d-b96f-a93fca4a3c45\"}],\"packageUris\":[\"http://schema.mathworks.com/mf0/Connector/R2020b\"],\"version\":\"1.0\"}"
  Thermal Monitoring & Assessment : Subsystem
      settings: PortSchema="{\"entries\":[{\"content\":{\"headerSize\":26,\"margin\":15,\"minimumSpacing\":25,\"sides\":[{\"content\":{\"connectorIds\":[\"In1\",\"In2\",\"In3\",\"In4\",\"LConn1\"]},\"type\":\"ConnectorPlacement.EquallySpacedRectSide\",\"uuid\":\"e0cfb70a-2480-46ad-8838-78efdb61b60e\"},{\"content\":{\"connectorIds\":[\"Out1\",\"Out2\",\"Out3\",\"Out4\"],\"side\":\"RIGHT\"},\"type\":\"ConnectorPlacement.EquallySpacedRectSide\",\"uuid\":\"0844e172-3ed8-42bd-94dc-a51d08e37039\"},{\"content\":{\"side\":\"TOP\"},\"type\":\"ConnectorPlacement.EquallySpacedRectSide\",\"uuid\":\"2415ea6e-ae7d-422f-a1cc-5a10cd0c87f7\"}]},\"type\":\"ConnectorPlacement.EquallySpacedConnector\",\"uuid\":\"814347a2-9201-4b2d-b96f-a93fca4a3c45\"}],\"packageUris\":[\"http://schema.mathworks.com/mf0/Connector/R2020b\"],\"version\":\"1.0\"}"
  IF-BTP-PRS-01 : PMIOPort  Side=Right  ConnectionType=Bus: ThermalNetwork
  IF-STP-PRS-01 : PMIOPort  Port=2  Side=Right  ConnectionType=Bus: ThermalNetwork
  IF-TBI-PRS-01 : PMIOPort  Port=3  Side=Right  ConnectionType=Bus: ThermalNetwork
  IF-PWR-TMS-01 : PMIOPort  Port=4  Side=Left  ConnectionType=Bus: ElectricalPower
  Bus Element Out1 : Outport  PortName=IF-TMS-GNC-01
  Bus Element Out2 : Outport  Port=2  PortName=IF-TMS-BTA-01
  Bus Element Out3 : Outport  Port=3  PortName=IF-TMS-STA-01
  Bus Element Out4 : Outport  Port=4  PortName=IF-TMS-SAF-01
  wires:
  Super Heavy Thermal Protection/3(IF-BTP-LOC-TBI-STP-01) -> Thermal Barriers & Discontinuity Protection/1(IF-BTP-LOC-TBI-STP-01)
  Bus Element In2/1 -> Super Heavy Thermal Protection/2(IF-ATM-BTP-01)
  Bus Element In3/1 -> Super Heavy Thermal Protection/1(IF-BNZ-BTP-01)
  Super Heavy Thermal Protection/1(IF-BTP-ACR-TBI-GAP-01) -> Thermal Barriers & Discontinuity Protection/3(IF-BTP-ACR-TBI-GAP-01)
  Bus Element In1/1 -> Ship Primary TPS/2(IF-ATM-STP-01)
  Bus Element In4/1 -> Ship Primary TPS/1(IF-SNZ-STP-01)
  Super Heavy Thermal Protection/2(IF-BTP-FHI-TBI-INT-01) -> Thermal Barriers & Discontinuity Protection/2(IF-BTP-FHI-TBI-INT-01)
  Ship Primary TPS/1(IF-STP-ACR-TBI-GAP-01) -> Thermal Barriers & Discontinuity Protection/6(IF-STP-ACR-TBI-GAP-01)
  Ship Primary TPS/2(IF-STP-CTL-TBI-CTL-01) -> Thermal Barriers & Discontinuity Protection/5(IF-STP-CTL-TBI-CTL-01)
  Ship Primary TPS/3(IF-STP-LOC-TBI-STP-01) -> Thermal Barriers & Discontinuity Protection/4(IF-STP-LOC-TBI-STP-01)
  Thermal Barriers & Discontinuity Protection/1(IF-TBI-GAP-TMS-SNS-01) -> Thermal Monitoring & Assessment/1(IF-TBI-GAP-TMS-SNS-01)
  Thermal Barriers & Discontinuity Protection/2(IF-TBI-INT-TMS-SNS-01) -> Thermal Monitoring & Assessment/2(IF-TBI-INT-TMS-SNS-01)
  Bus Element In5/1 -> Thermal Monitoring & Assessment/4(IF-GNC-TMS-01)
  Thermal Barriers & Discontinuity Protection/3(IF-TBI-CTL-TMS-SNS-01) -> Thermal Monitoring & Assessment/3(IF-TBI-CTL-TMS-SNS-01)
  Thermal Monitoring & Assessment/1(IF-TMS-GNC-01) -> Bus Element Out1/1
  Thermal Monitoring & Assessment/2(IF-TMS-BTA-01) -> Bus Element Out2/1
  Thermal Monitoring & Assessment/3(IF-TMS-STA-01) -> Bus Element Out3/1
  Thermal Monitoring & Assessment/4(IF-TMS-SAF-01) -> Bus Element Out4/1
  connections:
  Ship Primary TPS/RConn1 -- IF-STP-PRS-01/RConn1
  Super Heavy Thermal Protection/RConn1 -- IF-BTP-PRS-01/RConn1
  Thermal Barriers & Discontinuity Protection/RConn1 -- IF-TBI-PRS-01/RConn1
  IF-PWR-TMS-01/RConn1 -- Thermal Monitoring & Assessment/LConn1

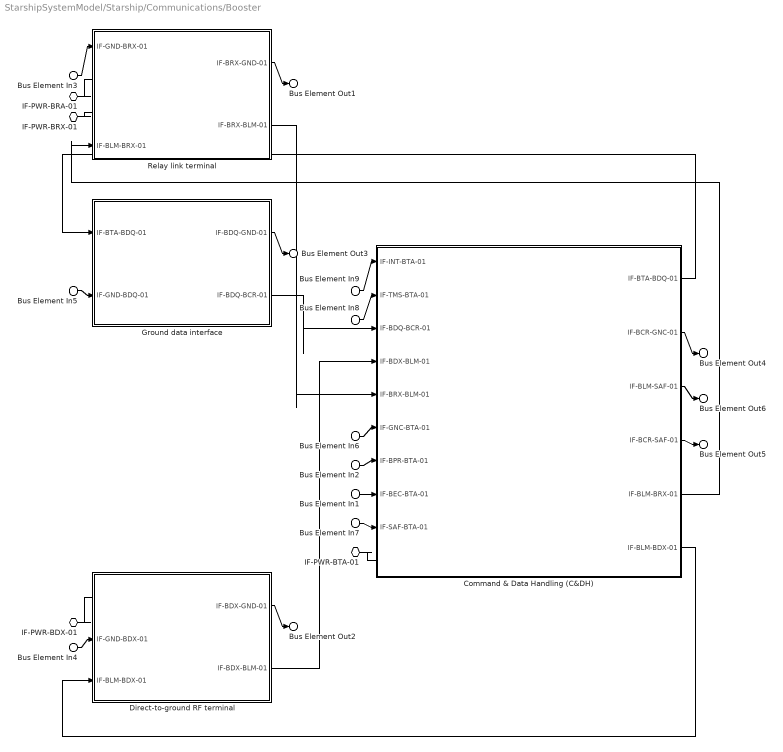
== system StarshipSystemModel/Starship/Communications/Booster ==
  Bus Element In9 : Inport  PortName=IF-INT-BTA-01
  Bus Element In8 : Inport  Port=2  PortName=IF-TMS-BTA-01
  Bus Element In6 : Inport  Port=3  PortName=IF-GNC-BTA-01
  Bus Element In2 : Inport  Port=4  PortName=IF-BPR-BTA-01
  Bus Element In1 : Inport  Port=5  PortName=IF-BEC-BTA-01
  Bus Element In3 : Inport  Port=6  PortName=IF-GND-BRX-01
  Bus Element In4 : Inport  Port=7  PortName=IF-GND-BDX-01
  Bus Element In5 : Inport  Port=8  PortName=IF-GND-BDQ-01
  Bus Element In7 : Inport  Port=9  PortName=IF-SAF-BTA-01
  Command & Data Handling (C&DH) : Subsystem
      settings: PortSchema="{\"entries\":[{\"content\":{\"headerSize\":26,\"margin\":15,\"minimumSpacing\":25,\"sides\":[{\"content\":{\"connectorIds\":[\"In1\",\"In2\",\"In3\",\"In4\",\"In5\",\"In6\",\"In7\",\"In8\",\"In9\",\"LConn1\"]},\"type\":\"ConnectorPlacement.EquallySpacedRectSide\",\"uuid\":\"57d8a002-ec9a-4125-b797-7e7c6712bf02\"},{\"content\":{\"connectorIds\":[\"Out1\",\"Out2\",\"Out3\",\"Out4\",\"Out5\",\"Out6\"],\"side\":\"RIGHT\"},\"type\":\"ConnectorPlacement.EquallySpacedRectSide\",\"uuid\":\"9c166a96-12fc-4382-8ebe-da88da7fda26\"},{\"content\":{\"side\":\"TOP\"},\"type\":\"ConnectorPlacement.EquallySpacedRectSide\",\"uuid\":\"d709cb41-f5aa-4a2a-ad2b-35894222a9c1\"}]},\"type\":\"ConnectorPlacement.EquallySpacedConnector\",\"uuid\":\"04bb3772-118b-42d1-ac15-43c1b901053a\"}],\"packageUris\":[\"http://schema.mathworks.com/mf0/Connector/R2020b\"],\"version\":\"1.0\"}"
  Direct-to-ground RF terminal : Subsystem
      settings: PortSchema="{\"entries\":[{\"content\":{\"headerSize\":26,\"margin\":15,\"minimumSpacing\":25,\"sides\":[{\"content\":{\"connectorIds\":[\"LConn1\",\"In1\",\"In2\"]},\"type\":\"ConnectorPlacement.EquallySpacedRectSide\",\"uuid\":\"57d8a002-ec9a-4125-b797-7e7c6712bf02\"},{\"content\":{\"connectorIds\":[\"Out1\",\"Out2\"],\"side\":\"RIGHT\"},\"type\":\"ConnectorPlacement.EquallySpacedRectSide\",\"uuid\":\"9c166a96-12fc-4382-8ebe-da88da7fda26\"},{\"content\":{\"side\":\"TOP\"},\"type\":\"ConnectorPlacement.EquallySpacedRectSide\",\"uuid\":\"d709cb41-f5aa-4a2a-ad2b-35894222a9c1\"}]},\"type\":\"ConnectorPlacement.EquallySpacedConnector\",\"uuid\":\"04bb3772-118b-42d1-ac15-43c1b901053a\"}],\"packageUris\":[\"http://schema.mathworks.com/mf0/Connector/R2020b\"],\"version\":\"1.0\"}"
  Ground data interface : Subsystem
      settings: PortSchema="{\"entries\":[{\"content\":{\"headerSize\":26,\"margin\":15,\"minimumSpacing\":25,\"sides\":[{\"content\":{\"connectorIds\":[\"In1\",\"In2\"]},\"type\":\"ConnectorPlacement.EquallySpacedRectSide\",\"uuid\":\"57d8a002-ec9a-4125-b797-7e7c6712bf02\"},{\"content\":{\"connectorIds\":[\"Out1\",\"Out2\"],\"side\":\"RIGHT\"},\"type\":\"ConnectorPlacement.EquallySpacedRectSide\",\"uuid\":\"9c166a96-12fc-4382-8ebe-da88da7fda26\"},{\"content\":{\"side\":\"TOP\"},\"type\":\"ConnectorPlacement.EquallySpacedRectSide\",\"uuid\":\"d709cb41-f5aa-4a2a-ad2b-35894222a9c1\"}]},\"type\":\"ConnectorPlacement.EquallySpacedConnector\",\"uuid\":\"04bb3772-118b-42d1-ac15-43c1b901053a\"}],\"packageUris\":[\"http://schema.mathworks.com/mf0/Connector/R2020b\"],\"version\":\"1.0\"}"
  Relay link terminal : Subsystem
      settings: PortSchema="{\"entries\":[{\"content\":{\"headerSize\":26,\"margin\":15,\"minimumSpacing\":25,\"sides\":[{\"content\":{\"connectorIds\":[\"In1\",\"LConn1\",\"LConn2\",\"In2\"]},\"type\":\"ConnectorPlacement.EquallySpacedRectSide\",\"uuid\":\"57d8a002-ec9a-4125-b797-7e7c6712bf02\"},{\"content\":{\"connectorIds\":[\"Out1\",\"Out2\"],\"side\":\"RIGHT\"},\"type\":\"ConnectorPlacement.EquallySpacedRectSide\",\"uuid\":\"9c166a96-12fc-4382-8ebe-da88da7fda26\"},{\"content\":{\"side\":\"TOP\"},\"type\":\"ConnectorPlacement.EquallySpacedRectSide\",\"uuid\":\"d709cb41-f5aa-4a2a-ad2b-35894222a9c1\"}]},\"type\":\"ConnectorPlacement.EquallySpacedConnector\",\"uuid\":\"04bb3772-118b-42d1-ac15-43c1b901053a\"}],\"packageUris\":[\"http://schema.mathworks.com/mf0/Connector/R2020b\"],\"version\":\"1.0\"}"
  IF-PWR-BRA-01 : PMIOPort  Side=Left  ConnectionType=Bus: ElectricalPower
  IF-PWR-BRX-01 : PMIOPort  Port=2  Side=Left  ConnectionType=Bus: ElectricalPower
  IF-PWR-BDX-01 : PMIOPort  Port=3  Side=Left  ConnectionType=Bus: ElectricalPower
  IF-PWR-BTA-01 : PMIOPort  Port=4  Side=Left  ConnectionType=Bus: ElectricalPower
  Bus Element Out2 : Outport  PortName=IF-BDX-GND-01
  Bus Element Out1 : Outport  Port=2  PortName=IF-BRX-GND-01
  Bus Element Out3 : Outport  Port=3  PortName=IF-BDQ-GND-01
  Bus Element Out4 : Outport  Port=4  PortName=IF-BCR-GNC-01
  Bus Element Out5 : Outport  Port=5  PortName=IF-BCR-SAF-01
  Bus Element Out6 : Outport  Port=6  PortName=IF-BLM-SAF-01
  wires:
  Bus Element In1/1 -> Command & Data Handling (C&DH)/8(IF-BEC-BTA-01)
  Bus Element In6/1 -> Command & Data Handling (C&DH)/6(IF-GNC-BTA-01)
  Bus Element In4/1 -> Direct-to-ground RF terminal/1(IF-GND-BDX-01)
  Bus Element In2/1 -> Command & Data Handling (C&DH)/7(IF-BPR-BTA-01)
  Bus Element In3/1 -> Relay link terminal/1(IF-GND-BRX-01)
  Bus Element In5/1 -> Ground data interface/2(IF-GND-BDQ-01)
  Relay link terminal/2(IF-BRX-BLM-01) -> Command & Data Handling (C&DH)/5(IF-BRX-BLM-01)
  Relay link terminal/1(IF-BRX-GND-01) -> Bus Element Out1/1
  Ground data interface/1("IF-BDQ-GND-01\t") -> Bus Element Out3/1
  Ground data interface/2(IF-BDQ-BCR-01) -> Command & Data Handling (C&DH)/3(IF-BDQ-BCR-01)
  Command & Data Handling (C&DH)/2(IF-BCR-GNC-01) -> Bus Element Out4/1
  Bus Element In7/1 -> Command & Data Handling (C&DH)/9(IF-SAF-BTA-01)
  Direct-to-ground RF terminal/1(IF-BDX-GND-01) -> Bus Element Out2/1
  Direct-to-ground RF terminal/2(IF-BDX-BLM-01) -> Command & Data Handling (C&DH)/4(IF-BDX-BLM-01)
  Command & Data Handling (C&DH)/1(IF-BTA-BDQ-01) -> Ground data interface/1(IF-BTA-BDQ-01)
  Command & Data Handling (C&DH)/3(IF-BLM-SAF-01) -> Bus Element Out6/1
  Command & Data Handling (C&DH)/4(IF-BCR-SAF-01) -> Bus Element Out5/1
  Command & Data Handling (C&DH)/5(IF-BLM-BRX-01) -> Relay link terminal/2(IF-BLM-BRX-01)
  Command & Data Handling (C&DH)/6(IF-BLM-BDX-01) -> Direct-to-ground RF terminal/2(IF-BLM-BDX-01)
  Bus Element In8/1 -> Command & Data Handling (C&DH)/2(IF-TMS-BTA-01)
  Bus Element In9/1 -> Command & Data Handling (C&DH)/1(IF-INT-BTA-01)
  connections:
  IF-PWR-BRA-01/RConn1 -- Relay link terminal/LConn1
  IF-PWR-BRX-01/RConn1 -- Relay link terminal/LConn2
  IF-PWR-BDX-01/RConn1 -- Direct-to-ground RF terminal/LConn1
  IF-PWR-BTA-01/RConn1 -- Command & Data Handling (C&DH)/LConn1
